simulink model "fem_connection_w_matlab"  (R2026b)
settings: Solver=ode23s  StopTime=60  FixedStep=0.05  MaxStep=0.001
libraries: fl_lib x34, ee_lib x12, nesl_utility x8
settings Model: Creator=Theof  LastModifiedBy=Theof
settings SolverCC: MaxConsecutiveMinStep=20
settings SimscapeCC: SimscapeLogType=all  SimscapeNominalValues="[{\"value\":\"1\",\"unit\":\"A\"},{\"value\":\"1\",\"unit\":\"bar\"},{\"value\":\"1\",\"unit\":\"cm^2\"},{\"value\":\"1\",\"unit\":\"cm^3/s\"},{\"value\":\"1\",\"unit\":\"kJ/kg\"},{\"value\":\"1\",\"unit\":\"kW\"},{\"value\":\"1\",\"unit\":\"l\"},{\"value\":\"1\",\"unit\":\"N\"},{\"value\":\"1\",\"unit\":\"N*m\"},{\"value\":\"1\",\"unit\":\"V\"},{\"value\":\"0.001\",\"unit\":\"Wb\"}]"  SimscapeUseEnergyAccounting=off

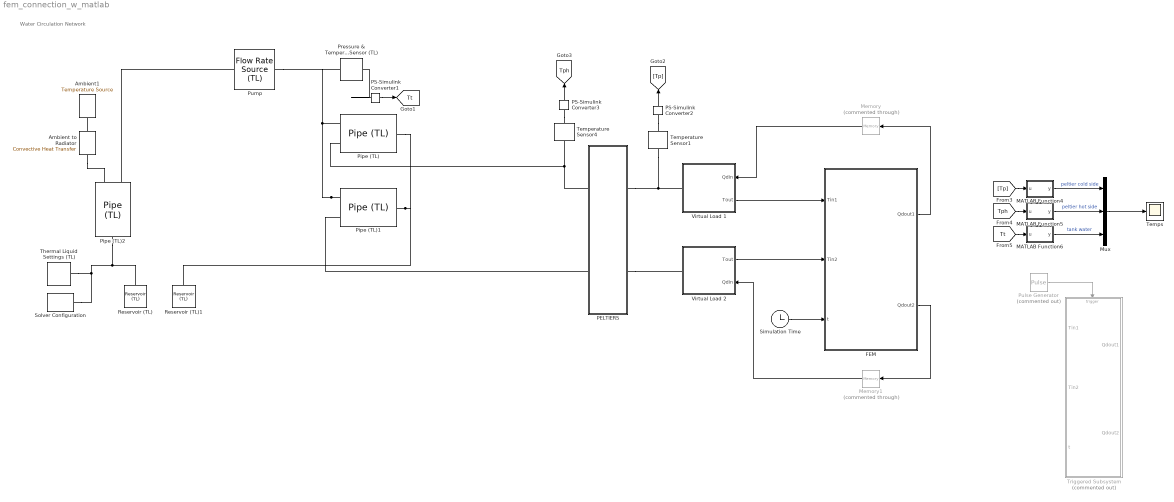
== system fem_connection_w_matlab ==
  note: Water Circulation Network
  Ambient to Radiator : fl_lib/Thermal/Thermal Elements/Convective Heat Transfer  thermal_type=foundation.enum.constant_variable.constant  area=15*25 cm^2  heat_tr_coeff=56 W/(K*m^2)  min_heat_tr_coeff=1e-3 W/(K*m^2)  T_specify=off  T_priority=None  T=0 K  T_nominal_specify=off  T_nominal_value=1  T_nominal_unit=K  Q_specify=off  Q_priority=None  Q=0 W  Q_nominal_specify=off  Q_nominal_value=1  Q_nominal_unit=W
  Ambient1 : fl_lib/Thermal/Thermal Sources/Temperature Source  temperature=30 degC
  FEM : MATLAB Function  InitFcn=|  TreatAsAtomicUnit=on
      | clear all;
      | close all;
      settings: MinAlgLoopOccurrences=on
  MATLAB Function4 : MATLAB Function  TreatAsAtomicUnit=on
  MATLAB Function5 : MATLAB Function  TreatAsAtomicUnit=on
  MATLAB Function6 : MATLAB Function  TreatAsAtomicUnit=on
  Memory : Memory  Commented=through
  Memory1 : Memory  Commented=through
  Mux : Mux  Inputs=3
  PELTIERS : Subsystem  mask{vpel=6, rpel=0.5}
      mask prompts: vpel "Voltage"; rpel "Series Resistor"
      mask DialogControl DescGroupVar Prompt: Peltier
  PS-Simulink Converter1 : nesl_utility/PS-Simulink Converter  PhysicalDomain=network_engine_domain  SubClassName=ps_output  LeftPortType=input  RightPortType=output  PseudoPeriodic=off  Frequencies=[]  VectorFormat=inherit  Unit=inherit  AffineConversion=off
  PS-Simulink Converter2 : nesl_utility/PS-Simulink Converter  PhysicalDomain=network_engine_domain  SubClassName=ps_output  LeftPortType=input  RightPortType=output  PseudoPeriodic=off  Frequencies=[]  VectorFormat=inherit  Unit=inherit  AffineConversion=off
  PS-Simulink Converter3 : nesl_utility/PS-Simulink Converter  PhysicalDomain=network_engine_domain  SubClassName=ps_output  LeftPortType=input  RightPortType=output  PseudoPeriodic=off  Frequencies=[]  VectorFormat=inherit  Unit=inherit  AffineConversion=off
  Pipe (TL) : fl_lib/Thermal Liquid/Elements/Pipe (TL)  length=0.5 m  area=4.2e-5 m^2  Dh=0.00175 m  length_add=1 m  roughness=15e-6 m  Re_lam=2000  Re_tur=4000  shape_factor=64  Nu_lam=3.66  dynamic_compressibility=true  inertia=false  p0=0.101325 MPa  T0=30 degC  mdot0=0 kg/s  p_nominal=0.101325 MPa  T_nominal=293.15 K
  Pipe (TL)1 : fl_lib/Thermal Liquid/Elements/Pipe (TL)  length=0.5 m  area=4.2e-5 m^2  Dh=0.00175 m  length_add=1 m  roughness=15e-6 m  Re_lam=2000  Re_tur=4000  shape_factor=64  Nu_lam=3.66  dynamic_compressibility=true  inertia=false  p0=0.101325 MPa  T0=30 degC  mdot0=0 kg/s  p_nominal=0.101325 MPa  T_nominal=293.15 K
  Pipe (TL)2 : fl_lib/Thermal Liquid/Elements/Pipe (TL)  length=3 m  area=4.2e-5 m^2  Dh=0.00175 m  length_add=1 m  roughness=15e-6 m  Re_lam=2000  Re_tur=4000  shape_factor=64  Nu_lam=3.66  dynamic_compressibility=true  inertia=false  p0=0.101325 MPa  T0=30 degC  mdot0=0 kg/s  p_nominal=0.101325 MPa  T_nominal=293.15 K
  Pressure & Temperature Sensor (TL) : fl_lib/Thermal Liquid/Sensors/Pressure & Temperature Sensor (TL)  reference=foundation.enum.MeasurementReference.absolute  pressure=false  pressure_spec=foundation.enum.PressureMeasementSpec.Absolute  temperature=true
  Pulse Generator : DiscretePulseGenerator  Commented=on  PulseType=Time based  Period=0.01  PulseWidth=50
  Pump : fl_lib/Thermal Liquid/Sources/Flow Rate Source (TL)  source_type=foundation.enum.constant_controlled.constant  flow_type=foundation.enum.mass_volumetric_flow.volumetric  mass_flow=0 kg/s  volumetric_flow=240/60 lpm  power_spec=foundation.enum.power_spec.none  area=8 mm^2
  Reservoir (TL) : fl_lib/Thermal Liquid/Elements/Reservoir (TL)  pressure_input=false  pressure_spec=foundation.enum.pressure_spec.atmospheric  reservoir_pressure=0.101325 MPa  temperature_input=false  reservoir_temperature=303 K  area=0.01 m^2  input_error_spec=foundation.enum.input_range_error.warn
  Reservoir (TL)1 : fl_lib/Thermal Liquid/Elements/Reservoir (TL)  pressure_input=false  pressure_spec=foundation.enum.pressure_spec.atmospheric  reservoir_pressure=0.101325 MPa  temperature_input=false  reservoir_temperature=303 K  area=0.01 m^2  input_error_spec=foundation.enum.input_range_error.warn
  Simulation Time : Clock
  Solver Configuration : nesl_utility/Solver Configuration  PhysicalDomain=network_engine_domain  SubClassName=solver  LeftPortType=input  RightPortType=generic  Tones=[]  Harmonics=[]  SimulateNoise=off  Profile=off  UseLocalSampling=off  EnableSwitchedLinearOptims=on  FrequencyDomain=off  UseCCode=off  RelTol=0.001  AbsTol=0.001  MinStep=1e-09  ToWorkspace=off  RevertToSquareIcSolve=off  NumHomotopyIterations=100  PhasorMode=off  PhasorModeNumHarmonics=1  ConsistencySolver=NEWTON_XTOL_AFTER_FTOL  CanonicalOrdering=UNORDERED  OptimizeIntermediates=UNOPTIMIZED  MulticoreSolverChoice=BACKWARD_EULER  IndexReductionMethod=DerivativeReplacement  DoDC=off  ResidualTolerance=1e-09  ConsistencyTolSource=GLOBAL  ConsistencyAbsTol=0.001  ConsistencyRelTol=0.001  ConsistencyTolFactor=0.001  UseLocalSolver=off  LocalSolverChoice=NE_BACKWARD_EULER_ADVANCER  ResolveIndetEquations=on  FunctionEvalNumThread=1  LocalSolverSampleTime=0.5  DoFixedCost=off  MaxNonlinIter=3  MaxModeIter=2  ComputeImpulses=off  ImpulseIterations=2  LinearAlgebra=auto  LinearAlgebraNumThread=0  EquationFormulation=NE_TIME_EF  DelaysMemoryBudget=1024  AutomaticFiltering=on  FilteringTimeConstant=0.001  PartitionStorageMethod=AS_NEEDED  PartitionMemoryBudget=1024  PartitionMethod=BALANCED  MultibodyUseLocalSolver=off  MultibodyLocalSolverChoice=ODE1  MultibodyLocalSolverSampleTime=0.001
  Temperature Sensor1 : fl_lib/Thermal/Thermal Sensors/Temperature Sensor  temperature_measure=foundation.enum.MeasurementReference.absolute
  Temperature Sensor4 : fl_lib/Thermal/Thermal Sensors/Temperature Sensor  temperature_measure=foundation.enum.MeasurementReference.absolute
  Temps : Scope
      settings: ActiveDisplayYMinimum=29.654024875616422  ActiveDisplayYMaximum=31.219503985249894
  Thermal Liquid Settings (TL) : fl_lib/Thermal Liquid/Utilities/Thermal Liquid Settings (TL)  table_dimensions=foundation.enum.table_dimensions_TL.two_dimensional  T_TLU=[273.1600 : 10 : 373.16]' K  p_TLU=[0.01, 0.1, 5 : 5 : 50] MPa  T_atm=293.15 K  p_atm=0.101325 MPa  pT_region_flag=foundation.enum.pT_region_TL.min_max  T_min=273.16 K  T_max=363.16 K  p_min=0.05 MPa  p_max=50 MPa  T_min_1D=273.16 K  T_max_1D=363.16 K  p_min_1D=0.05 MPa  p_max_1D=50 MPa  pT_validity_TLU=[1, 1, 1, 1, 1, 1, 1, 1, 1, 1, 1, 1; 1, 1, 1, 1, 1, 1, 1, 1, 1, 1, 1, 1; 1, 1, 1, 1, 1, 1, 1, 1, 1, 1, 1, 1; 1, 1, 1, 1, 1, 1, 1, 1, 1, 1, 1, 1; 1, 1, 1, 1, 1, 1, 1, 1, 1, 1, 1, 1; 0, 1, 1, 1, 1, 1, 1, 1, 1, 1, 1, 1; 0, 1, 1, 1, 1, 1, 1, 1, 1, 1, 1, 1; 0, 1, 1, 1, 1, 1, 1, 1, 1, 1, 1, 1; 0, 1, 1, 1, 1, 1, 1, 1, 1, 1, 1, 1; 0, 1, 1, 1, 1, 1, 1, 1, 1, 1, 1, 1; 0, 0, 1, 1, 1, 1, 1, 1, 1, 1, 1, 1]  properties_range_check=simscape.enum.assert.action.warn  rho_parameterization_2D=foundation.enum.rho_parameterization_2D.rho_beta_alpha  rho_parameterization_1D=foundation.enum.rho_parameterization_1D.rho_vector  rho_TLU=[999.7973, 999.8431, 1002.3216, 1004.8218, 1007.293, 1009.7358, 1012.1506, 1014.5379, 1016.8979, 1019.2311, 1021.538, 1023.8188; 999.6579, 999.7009, 1002.0303, 1004.382, 1006.7084, 1009.0101, 1011.2874, 1013.5407, 1015.7703, 1017.9766, 1020.1599, 1022.3206; 998.1632, 998.2045, 1000.4375, 1002.6924, 1004.9239, 1007.1324, 1009.3183, 1011.4819, 1013.6236, 1015.7438, 1017.8428, 1019.921; 995.6057, 995.6458, 997.8186, 1000.0128, 1002.1841, 1004.3332, 1006.4603, 1008.566, 1010.6505, 1012.7144, 1014.758, 1016.7815; 992.1724, 992.2119, 994.3513, 996.5113, 998.6484, 1000.7633, 1002.8563, 1004.928, 1006.9788, 1009.009, 1011.0192, 1013.0097; 988.02, 988.0299, 990.1568, 992.3035, 994.4268, 996.5273, 998.6056, 1000.6622, 1002.6976, 1004.7123, 1006.7067, 1008.6813; 983.18, 983.1901, 985.3217, 987.4721, 989.5983, 991.7008, 993.7803, 995.8374, 997.8726, 999.8864, 1001.8795, 1003.8522; 977.75, 977.7583, 979.9094, 982.0783, 984.2216, 986.34, 988.4343, 990.505, 992.5529, 994.5786, 996.5825, 998.5654; 971.77, 971.7836, 973.9673, 976.1678, 978.3409, 980.4876, 982.6087, 984.7049, 986.7768, 988.8254, 990.8511, 992.8545; 965.26, 965.3023, 967.5311, 969.7753, 971.9901, 974.1764, 976.3354, 978.4676, 980.5741, 982.6556, 984.7129, 986.7465; 958.62, 958.6315, 960.627, 962.9267, 965.1944, 967.4314, 969.6387, 971.8173, 973.9681, 976.0921, 978.19, 980.2628] kg/m^3  beta_TLU=[1.9649, 1.9654, 1.9929, 2.0213, 2.0499, 2.0787, 2.1078, 2.1372, 2.1668, 2.1966, 2.2268, 2.2572; 2.0913, 2.0918, 2.1191, 2.1471, 2.1752, 2.2036, 2.2322, 2.261, 2.2899, 2.3191, 2.3485, 2.3781; 2.1786, 2.1791, 2.2067, 2.235, 2.2634, 2.2919, 2.3206, 2.3494, 2.3784, 2.4075, 2.4367, 2.4661; 2.2332, 2.2337, 2.2619, 2.2908, 2.3197, 2.3487, 2.3778, 2.407, 2.4363, 2.4657, 2.4951, 2.5246; 2.26, 2.2605, 2.2895, 2.3191, 2.3487, 2.3784, 2.4081, 2.4378, 2.4675, 2.4973, 2.5272, 2.5571; 2.2638, 2.2638, 2.2936, 2.324, 2.3544, 2.3848, 2.4151, 2.4455, 2.4758, 2.5062, 2.5365, 2.5669; 2.2472, 2.2472, 2.2779, 2.3092, 2.3403, 2.3715, 2.4025, 2.4336, 2.4646, 2.4955, 2.5264, 2.5573; 2.214, 2.214, 2.2455, 2.2776, 2.3096, 2.3415, 2.3733, 2.405, 2.4367, 2.4683, 2.4998, 2.5313; 2.1668, 2.1668, 2.1992, 2.2321, 2.2649, 2.2976, 2.3301, 2.3626, 2.3949, 2.4272, 2.4593, 2.4914; 2.1081, 2.1081, 2.1413, 2.175, 2.2086, 2.2421, 2.2754, 2.3085, 2.3415, 2.3744, 2.4072, 2.4399; 2.0494, 2.0494, 2.0739, 2.1084, 2.1428, 2.177, 2.211, 2.2449, 2.2786, 2.3121, 2.3455, 2.3788] GPa  alpha_TLU=1e-4 * [-.679, -.676, -.49, -.307, -.13, .041, .206, .365, .519, .668, .811, .949; .878, .881, .998, 1.114, 1.227, 1.337, 1.445, 1.549, 1.651, 1.75, 1.846, 1.939; 2.068, 2.069, 2.141, 2.213, 2.283, 2.352, 2.42, 2.486, 2.551, 2.614, 2.676, 2.736; 3.034, 3.035, 3.074, 3.113, 3.152, 3.191, 3.229, 3.267, 3.305, 3.341, 3.377, 3.413; 3.855, 3.856, 3.87, 3.884, 3.899, 3.914, 3.93, 3.946, 3.961, 3.977, 3.993, 4.009; 4.578, 4.578, 4.572, 4.566, 4.562, 4.558, 4.555, 4.552, 4.55, 4.549, 4.548, 4.547; 5.233, 5.233, 5.209, 5.186, 5.165, 5.144, 5.125, 5.107, 5.09, 5.074, 5.059, 5.045; 5.84, 5.84, 5.801, 5.762, 5.725, 5.691, 5.657, 5.625, 5.595, 5.566, 5.538, 5.512; 6.414, 6.414, 6.36, 6.307, 6.256, 6.208, 6.161, 6.117, 6.074, 6.033, 5.994, 5.956; 6.967, 6.967, 6.898, 6.831, 6.766, 6.705, 6.646, 6.589, 6.535, 6.482, 6.432, 6.384; 7.519, 7.519, 7.423, 7.342, 7.264, 7.189, 7.118, 7.049, 6.983, 6.92, 6.859, 6.8] 1/K  rho_TLU_2=[999.7973, 999.8431, 1002.3216, 1004.8218, 1007.293, 1009.7358, 1012.1506, 1014.5379, 1016.8979, 1019.2311, 1021.538, 1023.8188; 999.6579, 999.7009, 1002.0303, 1004.382, 1006.7084, 1009.0101, 1011.2874, 1013.5407, 1015.7703, 1017.9766, 1020.1599, 1022.3206; 998.1632, 998.2045, 1000.4375, 1002.6924, 1004.9239, 1007.1324, 1009.3183, 1011.4819, 1013.6236, 1015.7438, 1017.8428, 1019.921; 995.6057, 995.6458, 997.81864, 1000.0128, 1002.1841, 1004.3332, 1006.4603, 1008.566, 1010.6505, 1012.7144, 1014.758, 1016.7815; 992.1724, 992.2119, 994.3513, 996.5113, 998.6484, 1000.7633, 1002.8563, 1004.928, 1006.9788, 1009.009, 1011.0192, 1013.0097; 988.02, 988.0299, 990.1568, 992.3035, 994.4268, 996.5273, 998.6056, 1000.6622, 1002.6976, 1004.7123, 1006.7067, 1008.6813; 983.18, 983.1901, 985.3217, 987.4721, 989.5983, 991.7008, 993.7803, 995.8374, 997.8726, 999.8864, 1001.8795, 1003.8522; 977.75, 977.7583, 979.9094, 982.0783, 984.2216, 986.34, 988.4343, 990.505, 992.5529, 994.5786, 996.5825, 998.5654; 971.77, 971.7836, 973.9673, 976.1678, 978.3409, 980.4876, 982.6087, 984.7049, 986.7768, 988.8254, 990.8511, 992.8545; 965.26, 965.3023, 967.5311, 969.7753, 971.9901, 974.1764, 976.3354, 978.4676, 980.5741, 982.6556, 984.7129, 986.7465; 958.62, 958.6315, 960.627, 962.9267, 965.1944, 967.4314, 969.6387, 971.8173, 973.9681, 976.0921, 978.19, 980.2628] kg/m^3  rho_ref_3=998.21 kg/m^3  T_ref_3=293.16 K  p_ref_3=0.101325 MPa  beta_const_3=2.1791 GPa  alpha_const_3=2.0691e-4 1/K  rho_TLU_4=[999.84; 999.7; 998.2; 995.65; 992.21; 988.03; 983.19; 977.76; 971.78; 965.3; 958.8] kg/m^3  beta_const_4=2.1791 GPa  p_ref_4=0.101325 MPa  rho_ref_5=998.21 kg/m^3  T_ref_5=293.16 K  p_ref_5=0.101325 MPa  beta_const_5=2.1791 GPa  alpha_const_5=2.0691e-4 1/K  u_parameterization_2D=foundation.enum.u_parameterization_2D.u_cp  u_parameterization_1D=foundation.enum.u_parameterization_1D.u  u_TLU=[.0002, .0018, .086, .1588, .219, .267, .3034, .3288, .3436, .3483, .3435, .3294; 42.062, 42.06, 41.935, 41.804, 41.668, 41.527, 41.382, 41.233, 41.081, 40.924, 40.763, 40.599; 83.953, 83.948, 83.651, 83.349, 83.049, 82.749, 82.451, 82.153, 81.856, 81.56, 81.265, 80.971; 125.77, 125.76, 125.31, 124.86, 124.41, 123.97, 123.53, 123.1, 122.68, 122.25, 121.84, 121.42; 167.57, 167.56, 166.96, 166.37, 165.79, 165.21, 164.65, 164.09, 163.54, 163, 162.46, 161.94; 209.36, 209.36, 208.63, 207.9, 207.19, 206.48, 205.79, 205.11, 204.45, 203.79, 203.14, 202.5; 251.19, 251.19, 250.33, 249.47, 248.62, 247.79, 246.98, 246.18, 245.39, 244.62, 243.86, 243.12; 293.06, 293.06, 292.07, 291.07, 290.1, 289.14, 288.2, 287.28, 286.38, 285.49, 284.62, 283.77; 334.99, 334.99, 333.86, 332.73, 331.63, 330.54, 329.48, 328.44, 327.41, 326.41, 325.43, 324.46; 377, 377, 375.73, 374.46, 373.22, 372, 370.81, 369.64, 368.5, 367.38, 366.27, 365.19; 419.01, 419.01, 417.69, 416.27, 414.89, 413.54, 412.21, 410.91, 409.64, 408.4, 407.17, 405.98] kJ/kg  cp_TLU=[4.2199, 4.2194, 4.1957, 4.1726, 4.1508, 4.13, 4.1103, 4.0916, 4.0738, 4.0569, 4.0408, 4.0254; 4.1955, 4.1951, 4.1769, 4.1592, 4.1422, 4.1259, 4.1103, 4.0954, 4.0812, 4.0676, 4.0545, 4.0421; 4.1843, 4.184, 4.169, 4.1543, 4.1401, 4.1264, 4.1133, 4.1007, 4.0885, 4.0768, 4.0656, 4.0548; 4.1801, 4.1798, 4.1667, 4.1538, 4.1413, 4.1293, 4.1177, 4.1064, 4.0956, 4.0851, 4.075, 4.0653; 4.1796, 4.1794, 4.1675, 4.1558, 4.1444, 4.1334, 4.1227, 4.1123, 4.1023, 4.0926, 4.0832, 4.0741; 4.1813, 4.1813, 4.1702, 4.1592, 4.1484, 4.138, 4.1279, 4.1181, 4.1086, 4.0993, 4.0903, 4.0816; 4.185, 4.185, 4.1742, 4.1636, 4.1532, 4.1432, 4.1334, 4.1239, 4.1146, 4.1056, 4.0969, 4.0884; 4.1901, 4.1901, 4.1795, 4.169, 4.1588, 4.1489, 4.1393, 4.1299, 4.1207, 4.1118, 4.1032, 4.0947; 4.1968, 4.1968, 4.1862, 4.1757, 4.1655, 4.1555, 4.1458, 4.1364, 4.1273, 4.1183, 4.1096, 4.1012; 4.2052, 4.2052, 4.1944, 4.1837, 4.1733, 4.1632, 4.1534, 4.1438, 4.1345, 4.1255, 4.1166, 4.108; 4.2136, 4.2136, 4.2045, 4.1935, 4.1828, 4.1724, 4.1623, 4.1524, 4.1429, 4.1335, 4.1245, 4.1157] kJ/(K*kg)  u_TLU_2=[.0002, .0018, .086, .1588, .219, .267, .3034, .3288, .3436, .3483, .3435, .3294; 42.062, 42.06, 41.935, 41.804, 41.668, 41.527, 41.382, 41.233, 41.081, 40.924, 40.763, 40.599; 83.953, 83.948, 83.651, 83.349, 83.049, 82.749, 82.451, 82.153, 81.856, 81.56, 81.265, 80.971; 125.77, 125.76, 125.31, 124.86, 124.41, 123.97, 123.53, 123.1, 122.68, 122.25, 121.84, 121.42; 167.57, 167.56, 166.96, 166.37, 165.79, 165.21, 164.65, 164.09, 163.54, 163, 162.46, 161.94; 209.36, 209.36, 208.63, 207.9, 207.19, 206.48, 205.79, 205.11, 204.45, 203.79, 203.14, 202.5; 251.19, 251.19, 250.33, 249.47, 248.62, 247.79, 246.98, 246.18, 245.39, 244.62, 243.86, 243.12; 293.06, 293.06, 292.07, 291.07, 290.1, 289.14, 288.2, 287.28, 286.38, 285.49, 284.62, 283.77; 334.99, 334.99, 333.86, 332.73, 331.63, 330.54, 329.48, 328.44, 327.41, 326.41, 325.43, 324.46; 377, 377, 375.73, 374.46, 373.22, 372, 370.81, 369.64, 368.5, 367.38, 366.27, 365.19; 419.01, 419.01, 417.69, 416.27, 414.89, 413.54, 412.21, 410.91, 409.64, 408.4, 407.17, 405.98] kJ/kg  cp_TLU_3=[4.2199, 4.2194, 4.1957, 4.1726, 4.1508, 4.13, 4.1103, 4.0916, 4.0738, 4.0569, 4.0408, 4.0254; 4.1955, 4.1951, 4.1769, 4.1592, 4.1422, 4.1259, 4.1103, 4.0954, 4.0812, 4.0676, 4.0545, 4.0421; 4.1843, 4.184, 4.169, 4.1543, 4.1401, 4.1264, 4.1133, 4.1007, 4.0885, 4.0768, 4.0656, 4.0548; 4.1801, 4.1798, 4.1667, 4.1538, 4.1413, 4.1293, 4.1177, 4.1064, 4.0956, 4.0851, 4.075, 4.0653; 4.1796, 4.1794, 4.1675, 4.1558, 4.1444, 4.1334, 4.1227, 4.1123, 4.1023, 4.0926, 4.0832, 4.0741; 4.1813, 4.1813, 4.1702, 4.1592, 4.1484, 4.138, 4.1279, 4.1181, 4.1086, 4.0993, 4.0903, 4.0816; 4.185, 4.185, 4.1742, 4.1636, 4.1532, 4.1432, 4.1334, 4.1239, 4.1146, 4.1056, 4.0969, 4.0884; 4.1901, 4.1901, 4.1795, 4.169, 4.1588, 4.1489, 4.1393, 4.1299, 4.1207, 4.1118, 4.1032, 4.0947; 4.1968, 4.1968, 4.1862, 4.1757, 4.1655, 4.1555, 4.1458, 4.1364, 4.1273, 4.1183, 4.1096, 4.1012; 4.2052, 4.2052, 4.1944, 4.1837, 4.1733, 4.1632, 4.1534, 4.1438, 4.1345, 4.1255, 4.1166, 4.108; 4.2136, 4.2136, 4.2045, 4.1935, 4.1828, 4.1724, 4.1623, 4.1524, 4.1429, 4.1335, 4.1245, 4.1157] kJ/(K*kg)  u_TLU_4=[.0018; 42.06; 83.948; 125.76; 167.56; 209.36; 251.19; 293.06; 334.99; 377; 418.01] kJ/kg  cp_TLU_5=[4.2199; 4.1955; 4.1843; 4.1801; 4.1796; 4.1813; 4.185; 4.1901; 4.1968; 4.2052; 4.2136] kJ/(K*kg)  nu_TLU=[1.7917, 1.7914, 1.7763, 1.7615, 1.7473, 1.7338, 1.7208, 1.7085, 1.6967, 1.6854, 1.6747, 1.6645; 1.3061, 1.3059, 1.2986, 1.2914, 1.2845, 1.2779, 1.2716, 1.2656, 1.2598, 1.2543, 1.2491, 1.2441; 1.0032, 1.0032, .9995, .9959, .9924, .9891, .9859, .9829, .9801, .9774, .9748, .9724; .8006, .8005, .7987, .797, .7953, .7937, .7922, .7908, .7894, .7881, .787, .7859; .6577, .6577, .657, .6562, .6555, .6548, .6543, .6537, .6532, .6528, .6523, .652; .553, .553, .5529, .5527, .5526, .5525, .5524, .5524, .5524, .5524, .5524, .5525; .4739, .4739, .4741, .4743, .4745, .4747, .475, .4753, .4755, .4758, .4762, .4765; .4127, .4127, .4131, .4135, .4139, .4143, .4148, .4152, .4157, .4162, .4167, .4172; .3643, .3643, .3648, .3654, .3659, .3665, .367, .3676, .3682, .3688, .3694, .37; .3254, .3254, .3261, .3267, .3273, .328, .3286, .3293, .3299, .3306, .3312, .3319; .2866, .2866, .2945, .2952, .2959, .2965, .2972, .2979, .2986, .2993, .3, .3007] mm^2/s  nu_TLU_2=[1.7917; 1.3061; 1.0032; .8006; .6577; .553; .4739; .4127; .3643; .3254; .2866] mm^2/s  k_TLU=[561.04, 561.09, 563.8, 566.56, 569.32, 572.08, 574.82, 577.54, 580.24, 582.92, 585.57, 588.18; 580.02, 580.07, 582.45, 584.88, 587.32, 589.75, 592.18, 594.61, 597.02, 599.42, 601.8, 604.16; 598.44, 598.48, 600.73, 603.03, 605.33, 607.64, 609.94, 612.24, 614.54, 616.82, 619.1, 621.36; 615.48, 615.52, 617.73, 620, 622.26, 624.54, 626.81, 629.07, 631.34, 633.6, 635.85, 638.09; 630.6, 630.64, 632.87, 635.15, 637.44, 639.72, 642.01, 644.29, 646.57, 648.84, 651.11, 653.36; 643.61, 643.61, 645.88, 648.21, 650.53, 652.86, 655.18, 657.51, 659.82, 662.14, 664.44, 666.74; 654.39, 654.39, 656.73, 659.12, 661.5, 663.89, 666.27, 668.65, 671.02, 673.38, 675.74, 678.09; 663.13, 663.13, 665.54, 668, 670.46, 672.91, 675.36, 677.8, 680.24, 682.67, 685.09, 687.5; 670.02, 670.02, 672.51, 675.05, 677.59, 680.12, 682.64, 685.16, 687.67, 690.17, 692.66, 695.14; 675.27, 675.27, 677.85, 680.48, 683.11, 685.73, 688.34, 690.94, 693.53, 696.11, 698.68, 701.24; 680.52, 680.52, 681.77, 684.5, 687.22, 689.94, 692.64, 695.34, 698.02, 700.69, 703.35, 706] mW/(K*m)  k_TLU_2=[561.04; 580.02; 598.44; 615.48; 630.6; 643.61; 654.39; 663.13; 670.02; 675.27; 680.52] mW/(K*m)  air_fraction=0  R_air=0.287 kJ/(K*kg)  air_dissolution_model=false  p_crit=3 MPa
  Triggered Subsystem : Subsystem  Commented=on  TreatAsAtomicUnit=on
  Virtual Load 1 : Subsystem
      settings: PortSchema="{\"entries\":[{\"content\":{\"sides\":[{\"content\":{\"connectorIds\":[\"LConn1\"]},\"type\":\"ConnectorPlacement.EquallySpacedRectSide\",\"uuid\":\"79759e96-5e57-4a85-b619-76e876053b0b\"},{\"content\":{\"connectorIds\":[\"In1\",\"Out1\"],\"side\":\"RIGHT\"},\"type\":\"ConnectorPlacement.EquallySpacedRectSide\",\"uuid\":\"bcb97bc2-2e04-4b91-9910-82fec75ca7b9\"},{\"content\":{\"side\":\"TOP\"},\"type\":\"ConnectorPlacement.EquallySpacedRectSide\",\"uuid\":\"ac990c0e-cc9d-4775-92c6-a224dc339378\"}]},\"type\":\"ConnectorPlacement.EquallySpacedConnector\",\"uuid\":\"79859a5f-a68d-4327-a4da-875c33a15e27\"}],\"packageUris\":[\"http://schema.mathworks.com/mf0/Connector/R2020b\"],\"version\":\"1.0\"}"
  Virtual Load 2 : Subsystem
      settings: PortSchema="{\"entries\":[{\"content\":{\"sides\":[{\"content\":{\"connectorIds\":[\"LConn1\"]},\"type\":\"ConnectorPlacement.EquallySpacedRectSide\",\"uuid\":\"79759e96-5e57-4a85-b619-76e876053b0b\"},{\"content\":{\"connectorIds\":[\"In1\",\"Out1\"],\"side\":\"RIGHT\"},\"type\":\"ConnectorPlacement.EquallySpacedRectSide\",\"uuid\":\"bcb97bc2-2e04-4b91-9910-82fec75ca7b9\"},{\"content\":{\"side\":\"TOP\"},\"type\":\"ConnectorPlacement.EquallySpacedRectSide\",\"uuid\":\"ac990c0e-cc9d-4775-92c6-a224dc339378\"}]},\"type\":\"ConnectorPlacement.EquallySpacedConnector\",\"uuid\":\"79859a5f-a68d-4327-a4da-875c33a15e27\"}],\"packageUris\":[\"http://schema.mathworks.com/mf0/Connector/R2020b\"],\"version\":\"1.0\"}"
  tag scope: Tph=global, Tt=global
  wires:
  PS-Simulink Converter1/1 -> [Tt]
  PS-Simulink Converter3/1 -> [Tph]
  Virtual Load 2/1(Tout) -> FEM/2(Tin2)
  [Tt] -> MATLAB Function6/1(u)
  [Tp] -> MATLAB Function4/1(u)
  MATLAB Function4/1(y) -> Mux/1  "peltier cold side"
  MATLAB Function6/1(y) -> Mux/3  "tank water"
  [Tph] -> MATLAB Function5/1(u)
  Mux/1 -> Temps/1
  MATLAB Function5/1(y) -> Mux/2  "peltier hot side"
  PS-Simulink Converter2/1 -> [Tp]
  Simulation Time/1 -> FEM/3(t)
  Virtual Load 1/1(Tout) -> FEM/1(Tin1)
  Pulse Generator/1 -> Triggered Subsystem/Trigger
  FEM/1(Qdout1) -> Memory/1
  FEM/2(Qdout2) -> Memory1/1
  Memory/1 -> Virtual Load 1/1(Qdin)
  Memory1/1 -> Virtual Load 2/1(Qdin)
  connections:
  PELTIERS/LConn1 -- Pipe (TL)/LConn2 -- Temperature Sensor4/LConn1
  Pipe (TL)1/RConn1 -- Reservoir (TL)1/LConn1 -- Pipe (TL)/RConn1
  Thermal Liquid Settings (TL)/RConn1 -- Reservoir (TL)/LConn1 -- Pipe (TL)2/RConn1 -- Solver Configuration/RConn1
  Pipe (TL)1/LConn1 -- Pipe (TL)/LConn1 -- Pressure & Temperature Sensor (TL)/LConn1 -- Pump/RConn1
  PS-Simulink Converter3/LConn1 -- Temperature Sensor4/RConn1
  Ambient to Radiator/LConn1 -- Ambient1/LConn1
  PS-Simulink Converter1/LConn1 -- Pressure & Temperature Sensor (TL)/RConn1
  Ambient to Radiator/RConn1 -- Pipe (TL)2/LConn2
  Virtual Load 1/LConn1 -- PELTIERS/RConn1 -- Temperature Sensor1/LConn1
  PELTIERS/RConn2 -- Virtual Load 2/LConn1
  PS-Simulink Converter2/LConn1 -- Temperature Sensor1/RConn1
  Pipe (TL)2/LConn1 -- Pump/LConn1
  PELTIERS/LConn2 -- Pipe (TL)1/LConn2

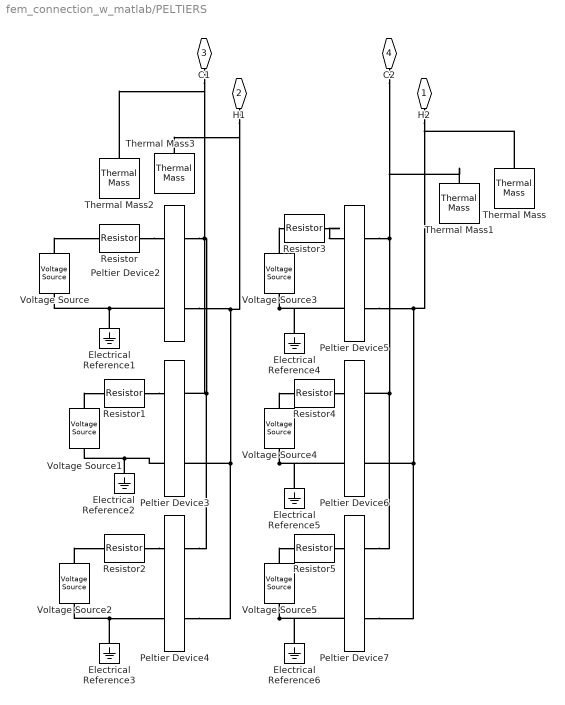
== system fem_connection_w_matlab/PELTIERS ==
  Electrical Reference{1..6} (6 alike) : fl_lib/Electrical/Electrical Elements/Electrical Reference
  Peltier Device{2..7} (6 alike) : ee_lib/Sensors & Transducers/Peltier Device  alpha=0.053 V/K  R=2 Ohm  K=1/2 W/K
  Resistor{,1..5} (6 alike) : fl_lib/Electrical/Electrical Elements/Resistor  R=rpel Ohm  i_specify=off  i_priority=None  i=0 A  i_nominal_specify=off  i_nominal_value=1  i_nominal_unit=A  v_specify=off  v_priority=None  v=0 V  v_nominal_specify=off  v_nominal_value=1  v_nominal_unit=V
  Thermal Mass{,1..3} (4 alike) : fl_lib/Thermal/Thermal Elements/Thermal Mass  mass_type=foundation.enum.constant_variable.constant  mass=(0.025/2)*3 kg  sp_heat=600 J/(K*kg)  mass_min=1e-6 kg  num_ports=foundation.enum.numPorts2.one  m_specify=off  m_priority=High  m=1 kg  m_nominal_specify=off  m_nominal_value=1  m_nominal_unit=kg  T_specify=on  T_priority=High  T=303 K  T_nominal_specify=off  T_nominal_value=1  T_nominal_unit=K  Q_specify=off  Q_priority=None  Q=0 W  Q_nominal_specify=off  Q_nominal_value=1  Q_nominal_unit=W
  Voltage Source : ee_lib/Sources/Voltage Source  dc_voltage=vpel V  ac_voltage=0 V  ac_shift=0 rad  ac_frequency=60 Hz  noise_mode=ee.enum.sources.noise.Disabled  PSD=0 V^2/Hz  sample_time=1e-3 s  repeatability=ee.enum.sources.repeatability.NotRepeatable  user_seed=0  auto_seed=3499211588  i_specify=off  i_priority=None  i=0 A  i_nominal_specify=off  i_nominal_value=1  i_nominal_unit=A  v_specify=off  v_priority=None  v=0 V  v_nominal_specify=off  v_nominal_value=1  v_nominal_unit=V
  Voltage Source1 : ee_lib/Sources/Voltage Source  dc_voltage=vpel V  ac_voltage=0 V  ac_shift=0 rad  ac_frequency=60 Hz  noise_mode=ee.enum.sources.noise.Disabled  PSD=0 V^2/Hz  sample_time=1e-3 s  repeatability=ee.enum.sources.repeatability.NotRepeatable  user_seed=0  auto_seed=3890346746  i_specify=off  i_priority=None  i=0 A  i_nominal_specify=off  i_nominal_value=1  i_nominal_unit=A  v_specify=off  v_priority=None  v=0 V  v_nominal_specify=off  v_nominal_value=1  v_nominal_unit=V
  Voltage Source2 : ee_lib/Sources/Voltage Source  dc_voltage=vpel V  ac_voltage=0 V  ac_shift=0 rad  ac_frequency=60 Hz  noise_mode=ee.enum.sources.noise.Disabled  PSD=0 V^2/Hz  sample_time=1e-3 s  repeatability=ee.enum.sources.repeatability.NotRepeatable  user_seed=0  auto_seed=545404223  i_specify=off  i_priority=None  i=0 A  i_nominal_specify=off  i_nominal_value=1  i_nominal_unit=A  v_specify=off  v_priority=None  v=0 V  v_nominal_specify=off  v_nominal_value=1  v_nominal_unit=V
  Voltage Source3 : ee_lib/Sources/Voltage Source  dc_voltage=vpel V  ac_voltage=0 V  ac_shift=0 rad  ac_frequency=60 Hz  noise_mode=ee.enum.sources.noise.Disabled  PSD=0 V^2/Hz  sample_time=1e-3 s  repeatability=ee.enum.sources.repeatability.NotRepeatable  user_seed=0  auto_seed=3922919431  i_specify=off  i_priority=None  i=0 A  i_nominal_specify=off  i_nominal_value=1  i_nominal_unit=A  v_specify=off  v_priority=None  v=0 V  v_nominal_specify=off  v_nominal_value=1  v_nominal_unit=V
  Voltage Source4 : ee_lib/Sources/Voltage Source  dc_voltage=vpel V  ac_voltage=0 V  ac_shift=0 rad  ac_frequency=60 Hz  noise_mode=ee.enum.sources.noise.Disabled  PSD=0 V^2/Hz  sample_time=1e-3 s  repeatability=ee.enum.sources.repeatability.NotRepeatable  user_seed=0  auto_seed=2715962282  i_specify=off  i_priority=None  i=0 A  i_nominal_specify=off  i_nominal_value=1  i_nominal_unit=A  v_specify=off  v_priority=None  v=0 V  v_nominal_specify=off  v_nominal_value=1  v_nominal_unit=V
  Voltage Source5 : ee_lib/Sources/Voltage Source  dc_voltage=vpel V  ac_voltage=0 V  ac_shift=0 rad  ac_frequency=60 Hz  noise_mode=ee.enum.sources.noise.Disabled  PSD=0 V^2/Hz  sample_time=1e-3 s  repeatability=ee.enum.sources.repeatability.NotRepeatable  user_seed=0  auto_seed=418932850  i_specify=off  i_priority=None  i=0 A  i_nominal_specify=off  i_nominal_value=1  i_nominal_unit=A  v_specify=off  v_priority=None  v=0 V  v_nominal_specify=off  v_nominal_value=1  v_nominal_unit=V
  H2 : PMIOPort  Side=Left
  H1 : PMIOPort  Port=2  Side=Left
  C1 : PMIOPort  Port=3  Side=Right
  C2 : PMIOPort  Port=4  Side=Right
  connections:
  Peltier Device7/RConn2 -- Peltier Device6/RConn2 -- Thermal Mass/LConn1 -- H2/RConn1 -- Peltier Device5/RConn2
  Peltier Device4/RConn1 -- Peltier Device3/RConn1 -- Thermal Mass2/LConn1 -- C1/RConn1 -- Peltier Device2/RConn1
  Peltier Device7/RConn1 -- Peltier Device6/RConn1 -- Thermal Mass1/LConn1 -- C2/RConn1 -- Peltier Device5/RConn1
  Peltier Device4/RConn2 -- Peltier Device3/RConn2 -- Thermal Mass3/LConn1 -- H1/RConn1 -- Peltier Device2/RConn2
  Electrical Reference1/LConn1 -- Voltage Source/RConn1 -- Peltier Device2/LConn2
  Electrical Reference2/LConn1 -- Peltier Device3/LConn2 -- Voltage Source1/RConn1
  Electrical Reference3/LConn1 -- Peltier Device4/LConn2 -- Voltage Source2/RConn1
  Voltage Source3/RConn1 -- Peltier Device5/LConn2 -- Electrical Reference4/LConn1
  Voltage Source4/RConn1 -- Peltier Device6/LConn2 -- Electrical Reference5/LConn1
  Voltage Source5/RConn1 -- Peltier Device7/LConn2 -- Electrical Reference6/LConn1
  Resistor/RConn1 -- Peltier Device2/LConn1
  Voltage Source/LConn1 -- Resistor/LConn1
  Resistor1/RConn1 -- Peltier Device3/LConn1
  Voltage Source1/LConn1 -- Resistor1/LConn1
  Resistor2/RConn1 -- Peltier Device4/LConn1
  Voltage Source2/LConn1 -- Resistor2/LConn1
  Voltage Source3/LConn1 -- Resistor3/LConn1
  Resistor3/RConn1 -- Peltier Device5/LConn1
  Voltage Source4/LConn1 -- Resistor4/LConn1
  Resistor4/RConn1 -- Peltier Device6/LConn1
  Resistor5/RConn1 -- Peltier Device7/LConn1
  Voltage Source5/LConn1 -- Resistor5/LConn1

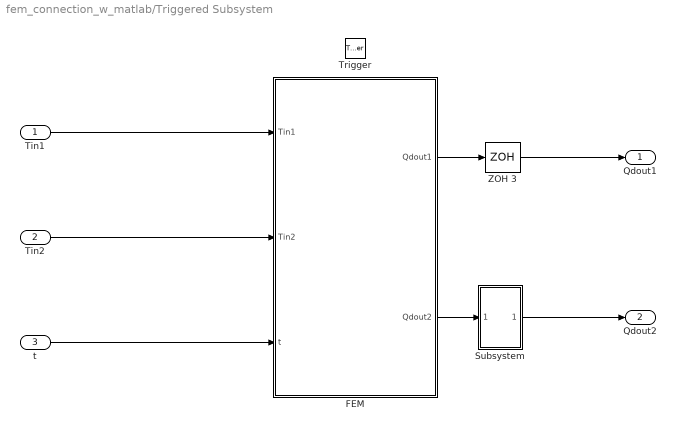
== system fem_connection_w_matlab/Triggered Subsystem ==
  Tin1 : Inport  LatchByDelayingOutsideSignal=on
  Tin2 : Inport  Port=2  LatchByDelayingOutsideSignal=on
  t : Inport  Port=3
  Trigger : TriggerPort  VariantControl=(inherit)
  FEM : MATLAB Function  InitFcn=|  TreatAsAtomicUnit=on
      | clear all;
      | close all;
  Subsystem : Subsystem
  ZOH 3 : ZeroOrderHold  SampleTime=-1
  Qdout1 : Outport
  Qdout2 : Outport  Port=2
  wires:
  FEM/1(Qdout1) -> ZOH 3/1
  Tin1/1 -> FEM/1(Tin1)
  Tin2/1 -> FEM/2(Tin2)
  ZOH 3/1 -> Qdout1/1
  t/1 -> FEM/3(t)
  FEM/2(Qdout2) -> Subsystem/1(In1)
  Subsystem/1(Out1) -> Qdout2/1

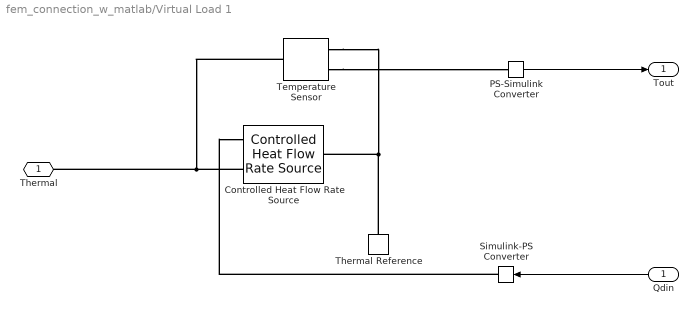
== system fem_connection_w_matlab/Virtual Load 1 ==
  Qdin : Inport
  Controlled Heat Flow Rate Source : fl_lib/Thermal/Thermal Sources/Controlled Heat Flow Rate Source
  PS-Simulink Converter : nesl_utility/PS-Simulink Converter  PhysicalDomain=network_engine_domain  SubClassName=ps_output  LeftPortType=input  RightPortType=output  PseudoPeriodic=off  Frequencies=[]  VectorFormat=inherit  Unit=inherit  AffineConversion=off
  Simulink-PS Converter : nesl_utility/Simulink-PS Converter  PhysicalDomain=network_engine_domain  SubClassName=ps_input  LeftPortType=input  RightPortType=output  PseudoPeriodic=off  Frequencies=[]  NoiseDistribution=none  NoiseParameters=[]  Unit=1  AffineConversion=off  FilteringAndDerivatives=provide  SimscapeFilterOrder=1  InputFilterTimeConstant=0.001  UdotUserProvided=0
  Temperature Sensor : fl_lib/Thermal/Thermal Sensors/Temperature Sensor  temperature_measure=foundation.enum.MeasurementReference.difference
  Thermal Reference : fl_lib/Thermal/Thermal Elements/Thermal Reference
  Thermal : PMIOPort  Side=Left
  Tout : Outport
  wires:
  PS-Simulink Converter/1 -> Tout/1
  Qdin/1 -> Simulink-PS Converter/1
  connections:
  Simulink-PS Converter/RConn1 -- Controlled Heat Flow Rate Source/RConn1
  Controlled Heat Flow Rate Source/RConn2 -- Temperature Sensor/LConn1 -- Thermal/RConn1
  Thermal Reference/LConn1 -- Temperature Sensor/RConn1 -- Controlled Heat Flow Rate Source/LConn1
  Temperature Sensor/RConn2 -- PS-Simulink Converter/LConn1

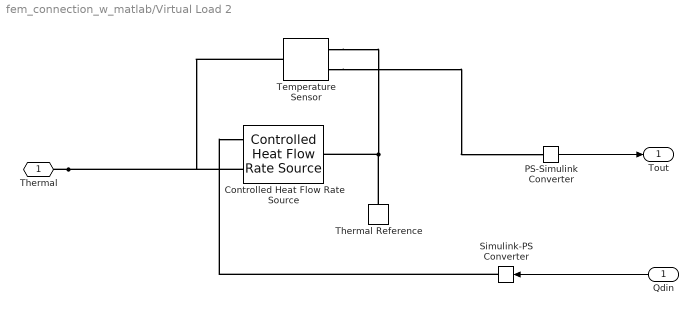
== system fem_connection_w_matlab/Virtual Load 2 ==
  Qdin : Inport
  Controlled Heat Flow Rate Source : fl_lib/Thermal/Thermal Sources/Controlled Heat Flow Rate Source
  PS-Simulink Converter : nesl_utility/PS-Simulink Converter  PhysicalDomain=network_engine_domain  SubClassName=ps_output  LeftPortType=input  RightPortType=output  PseudoPeriodic=off  Frequencies=[]  VectorFormat=inherit  Unit=inherit  AffineConversion=off
  Simulink-PS Converter : nesl_utility/Simulink-PS Converter  PhysicalDomain=network_engine_domain  SubClassName=ps_input  LeftPortType=input  RightPortType=output  PseudoPeriodic=off  Frequencies=[]  NoiseDistribution=none  NoiseParameters=[]  Unit=1  AffineConversion=off  FilteringAndDerivatives=provide  SimscapeFilterOrder=1  InputFilterTimeConstant=0.001  UdotUserProvided=0
  Temperature Sensor : fl_lib/Thermal/Thermal Sensors/Temperature Sensor  temperature_measure=foundation.enum.MeasurementReference.difference
  Thermal Reference : fl_lib/Thermal/Thermal Elements/Thermal Reference
  Thermal : PMIOPort  Side=Left
  Tout : Outport
  wires:
  PS-Simulink Converter/1 -> Tout/1
  Qdin/1 -> Simulink-PS Converter/1
  connections:
  Simulink-PS Converter/RConn1 -- Controlled Heat Flow Rate Source/RConn1
  Thermal/RConn1 -- Controlled Heat Flow Rate Source/RConn2 -- Temperature Sensor/LConn1
  Thermal Reference/LConn1 -- Controlled Heat Flow Rate Source/LConn1 -- Temperature Sensor/RConn1
  Temperature Sensor/RConn2 -- PS-Simulink Converter/LConn1

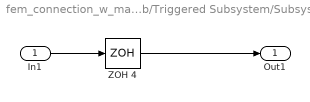
== system fem_connection_w_matlab/Triggered Subsystem/Subsystem ==
  In1 : Inport
  ZOH 4 : ZeroOrderHold  SampleTime=-1
  Out1 : Outport
  wires:
  In1/1 -> ZOH 4/1
  ZOH 4/1 -> Out1/1

== matlab function fem_connection_w_matlab/FEM ==
  settings: updateMethod=DISCRETE
  data: Qdout1 output; Tin1 input; Tin2 input; Qdout2 output; t input
function [Qdout1, Qdout2] = fcn(Tin1, Tin2, t)
    Qdout1 = 0.0;
    Qdout2 = 0.0;

    coder.extrinsic('model_m');
    
    %Qout = model_m(Tin1, Tin2, t); Qdout1 = Qout(1); Qdout2 = Qout(2);

    [Qdout1, Qdout2] = model_m(Tin1, Tin2, t);

end

== matlab function fem_connection_w_matlab/Triggered Subsystem/FEM ==
  settings: updateMethod=DISCRETE
  data: Qdout1 output; Tin1 input; Tin2 input; Qdout2 output; t input
function [Qdout1, Qdout2] = fcn(Tin1, Tin2, t)

    coder.extrinsic('model_m');
    
    Qdout1 = 0.0;
    Qdout2 = 0.0;
    
    %Qout = model_m(Tin1, Tin2, t); Qdout1 = Qout(1); Qdout2 = Qout(2);

    [Qdout1, Qdout2] = model_m(Tin1, Tin2, t);

end

== matlab function fem_connection_w_matlab/MATLAB Function4 ==
  data: u input; y output
function y = ktoc(u)

y = u-273;

== matlab function fem_connection_w_matlab/MATLAB Function5 ==
  data: u input; y output
function y = ktoc(u)

y = u-273;

== matlab function fem_connection_w_matlab/MATLAB Function6 ==
  data: u input; y output
function y = ktoc(u)

y = u-273;
